simulink model "Interleaved_Boost_Thevenin_Full_Control_ForDesign"  (R2024b)
settings: Solver=FixedStepAuto  StartTime=0.0  StopTime=5  MaxStep=1e-6  RelTol=1e-3
libraries: spsSeriesRLCBranchLib x6, spsCurrentMeasurementLib x5, spsMosfetLib x3, spsDiodeLib x2, spsVoltageMeasurementLib x2, spsDCVoltageSourceLib x1, sps_lib x1
settings Model: Creator=Parti  LastModifiedBy=Eng.Abd-Elrhman Saad

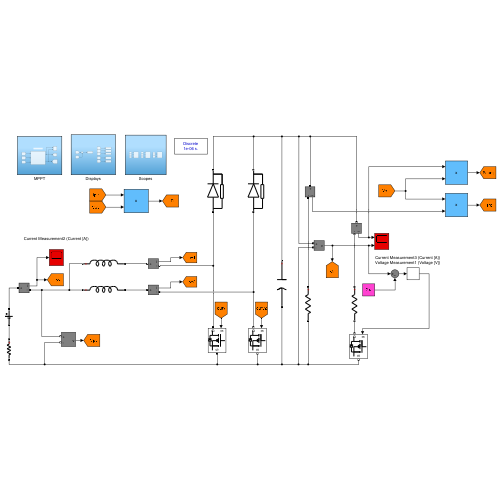
[thumbnail: Simulink's stored preview of the top-level diagram]
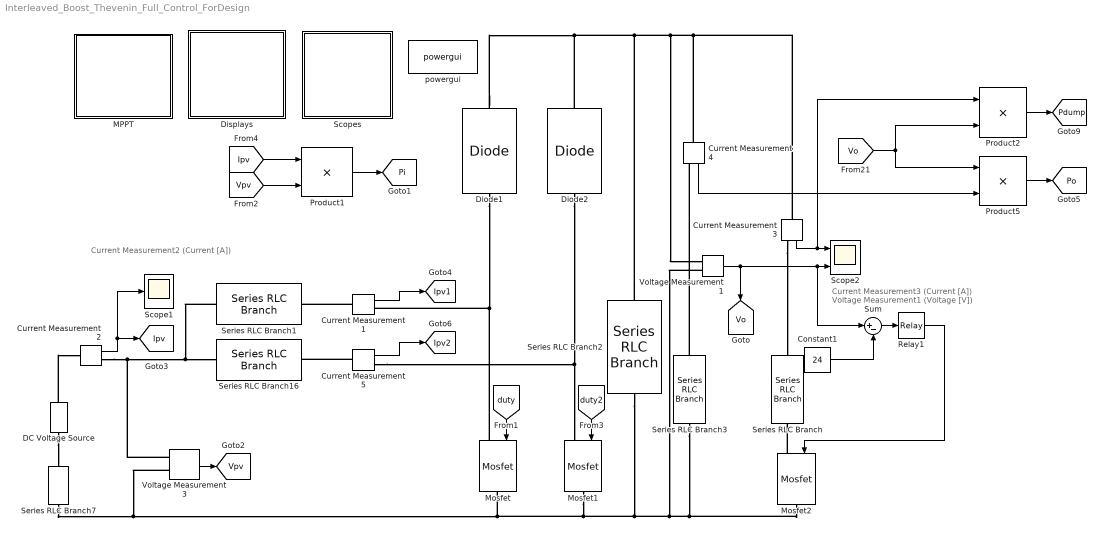
== system Interleaved_Boost_Thevenin_Full_Control_ForDesign ==
  note: Current Measurement2 (Current [A])
  note: Current Measurement3 (Current [A])
      | Voltage Measurement1 (Voltage [V])
  Constant1 : Constant  Value=24
  Current Measurement{1..5} (5 alike) : spsCurrentMeasurementLib/Current Measurement  PhasorSimulation=off  OutputType=Complex  PSBequivalent=0
  DC Voltage Source : spsDCVoltageSourceLib/DC Voltage Source  Amplitude=12  Measurements=None
  Diode1 : spsDiodeLib/Diode  Ron=0.001  Lon=0  Vf=0.8  IC=0  UseSnubber=0  Rs=500  Cs=250e-9  Measurements=off
  Diode2 : spsDiodeLib/Diode  Ron=0.001  Lon=0  Vf=0.8  IC=0  UseSnubber=0  Rs=500  Cs=250e-9  Measurements=off
  "Displays " : Subsystem
  MPPT : Subsystem
  Mosfet : spsMosfetLib/Mosfet  Ron=0.1  Lon=0  Rd=0.01  Vfd=0  IC=0  Rs=1e5  Cs=inf  Measurements=off
  Mosfet1 : spsMosfetLib/Mosfet  Ron=0.1  Lon=0  Rd=0.01  Vfd=0  IC=0  Rs=1e5  Cs=inf  Measurements=off
  Mosfet2 : spsMosfetLib/Mosfet  Ron=0.1  Lon=0  Rd=0.01  Vfd=0  IC=0  Rs=1e5  Cs=inf  Measurements=off
  Product1 : Product
  Product2 : Product
  Product5 : Product
  Relay1 : Relay  OnSwitchValue=0.5  OffSwitchValue=-0.5
  Scope1 : Scope
  Scope2 : Scope  NumInputPorts=2
  Scopes : Subsystem
  Series RLC Branch : spsSeriesRLCBranchLib/Series RLC Branch  LConnTagsString=__new0  RConnTagsString=__new0  BranchType=R  Resistance=57.6  Inductance=1e-3  SetiL0=off  InitialCurrent=0  Capacitance=1e-6  Setx0=off  InitialVoltage=0  Measurements=None
  Series RLC Branch1 : spsSeriesRLCBranchLib/Series RLC Branch  LConnTagsString=__new0  RConnTagsString=__new0  BranchType=L  Resistance=1  Inductance=2e-3  SetiL0=off  InitialCurrent=0  Capacitance=1000e-6  Setx0=on  InitialVoltage=100  Measurements=None
  Series RLC Branch16 : spsSeriesRLCBranchLib/Series RLC Branch  LConnTagsString=__new0  RConnTagsString=__new0  BranchType=L  Resistance=1  Inductance=2e-3  SetiL0=off  InitialCurrent=0  Capacitance=1000e-6  Setx0=on  InitialVoltage=100  Measurements=None
  Series RLC Branch2 : spsSeriesRLCBranchLib/Series RLC Branch  LConnTagsString=__new0  RConnTagsString=__new0  BranchType=C  Resistance=1  Inductance=1e-3  SetiL0=off  InitialCurrent=0  Capacitance=2e-3  Setx0=off  InitialVoltage=24  Measurements=None
  Series RLC Branch3 : spsSeriesRLCBranchLib/Series RLC Branch  LConnTagsString=__new0  RConnTagsString=__new0  BranchType=R  Resistance=220  Inductance=1e-3  SetiL0=off  InitialCurrent=0  Capacitance=1e-6  Setx0=off  InitialVoltage=0  Measurements=None
  Series RLC Branch7 : spsSeriesRLCBranchLib/Series RLC Branch  LConnTagsString=__new0  RConnTagsString=__new0  BranchType=R  Resistance=7  Inductance=1e-3  SetiL0=off  InitialCurrent=0  Capacitance=1e-6  Setx0=off  InitialVoltage=0  Measurements=None
  Sum : Sum  Inputs=|+-
  Voltage Measurement1 : spsVoltageMeasurementLib/Voltage Measurement  PhasorSimulation=off  OutputType=Complex  PSBequivalent=0
  Voltage Measurement3 : spsVoltageMeasurementLib/Voltage Measurement  PhasorSimulation=off  OutputType=Complex  PSBequivalent=0
  powergui : sps_lib/powergui  Priority=1  SimulationMode=Discrete  SampleTime=1e-6  frequency=60  Iterations=50  frequencyindice=0  Pbase=100e6  ErrMax=1e-4  UnitsV=kV  UnitsW=MW  buscounter=0  FunctionMessages=off  echomessages=off  EnableUseOfTLC=off  CurrentSourceSwitches=off  DisableSnubberDevices=off  DisableRonSwitches=off  DisableVfSwitches=off  DisplayEquations=off  AutomaticDiscreteSolvers=off  SolverType=Tustin/Backward Euler (TBE)  Interpol=off  ExternalGateDelay=off  methode=off  Ts=100  x0status=blocks  SPID=on  SwTol=0  HookPort=off  NonlinearTolerance=1e-4  nMaxIteration=100  ContinueOnMaxIteration=off  RestoreLinks=warning  ResistiveCurrentMeasurement=off  Frange=[0:2:500]  Ylog=off  Xlog=on  ShowGrid=off  save=off  variable=ZData  structure=0  ZoomFFT=off  StartTime=0.0  cycles=1  DisplayStyle=1  fundamental=60  FreqAxis=off  MaxFrequency=1000  frequencyindicesteady=1  RmsSteady=1  display=off
  tag scope: Ipv1=global, Ipv2=global, Ipv=global, Pdump=global, Pi=global, Po=global, Vo=global, Vpv=global
  wires:
  Current Measurement3/1 -> Product2/1, Scope2/1
  Voltage Measurement1/1 -> Scope2/2, Sum/1, [Vo]
  Current Measurement1/1 -> [Ipv1]
  Current Measurement5/1 -> [Ipv2]
  Constant1/1 -> Sum/2
  Sum/1 -> Relay1/1
  Relay1/1 -> Mosfet2/1
  [duty] -> Mosfet/1
  Voltage Measurement3/1 -> [Vpv]
  Current Measurement2/1 -> Scope1/1, [Ipv]
  [Ipv] -> Product1/1
  Product5/1 -> [Po]
  [Vpv] -> Product1/2
  Product1/1 -> [Pi]
  Current Measurement4/1 -> Product5/2
  Product2/1 -> [Pdump]
  [Vo] -> Product5/1, Product2/2
  [duty2] -> Mosfet1/1
  connections:
  Current Measurement5/LConn1 -- Series RLC Branch16/RConn1
  Diode1/RConn1 -- Current Measurement4/LConn1 -- Current Measurement3/LConn1 -- Voltage Measurement1/LConn1 -- Series RLC Branch2/LConn1 -- Diode2/RConn1
  Series RLC Branch2/RConn1 -- Mosfet2/RConn1 -- Series RLC Branch3/RConn1 -- Voltage Measurement1/LConn2 -- Mosfet1/RConn1 -- Series RLC Branch7/RConn1 -- Voltage Measurement3/LConn2 -- Mosfet/RConn1
  DC Voltage Source/RConn1 -- Current Measurement2/LConn1
  Current Measurement2/RConn1 -- Voltage Measurement3/LConn1 -- Series RLC Branch1/LConn1 -- Series RLC Branch16/LConn1
  Current Measurement3/RConn1 -- Series RLC Branch/LConn1
  Diode2/LConn1 -- Current Measurement5/RConn1 -- Mosfet1/LConn1
  Current Measurement1/LConn1 -- Series RLC Branch1/RConn1
  Diode1/LConn1 -- Mosfet/LConn1 -- Current Measurement1/RConn1
  Mosfet2/LConn1 -- Series RLC Branch/RConn1
  DC Voltage Source/LConn1 -- Series RLC Branch7/LConn1
  Series RLC Branch3/LConn1 -- Current Measurement4/RConn1

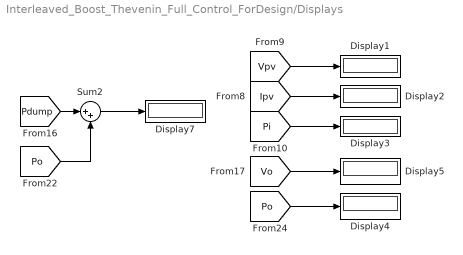
== system Interleaved_Boost_Thevenin_Full_Control_ForDesign/Displays  ==
  Display{1..5,7} (6 alike) : Display
  Sum2 : Sum  Inputs=|++
  wires:
  Sum2/1 -> Display7/1
  [Pi] -> Display3/1
  [Pdump] -> Sum2/1
  [Po] -> Display4/1
  [Po] -> Sum2/2
  [Ipv] -> Display2/1
  [Vpv] -> Display1/1
  [Vo] -> Display5/1

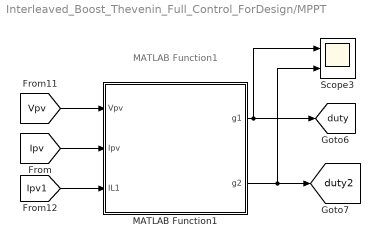
== system Interleaved_Boost_Thevenin_Full_Control_ForDesign/MPPT ==
  note: MATLAB Function1
  MATLAB Function1 : MATLAB Function  TreatAsAtomicUnit=on
  Scope3 : Scope  NumInputPorts=2
  tag scope: duty2=global, duty=global
  wires:
  [Ipv1] -> MATLAB Function1/3(IL1)
  [Ipv] -> MATLAB Function1/2(Ipv)
  MATLAB Function1/1(g1) -> Scope3/1, [duty]
  MATLAB Function1/2(g2) -> Scope3/2, [duty2]
  [Vpv] -> MATLAB Function1/1(Vpv)

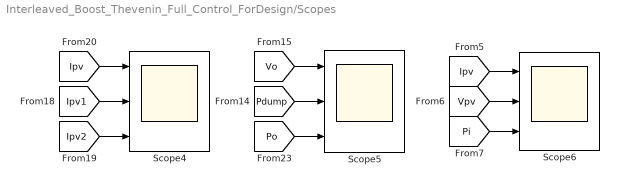
== system Interleaved_Boost_Thevenin_Full_Control_ForDesign/Scopes ==
  Scope4 : Scope  NumInputPorts=3
  Scope5 : Scope  NumInputPorts=3
  Scope6 : Scope  NumInputPorts=3
  wires:
  [Ipv1] -> Scope4/2
  [Vo] -> Scope5/1
  [Po] -> Scope5/3
  [Pdump] -> Scope5/2
  [Ipv] -> Scope6/1
  [Ipv2] -> Scope4/3
  [Ipv] -> Scope4/1
  [Pi] -> Scope6/3
  [Vpv] -> Scope6/2

== matlab function Interleaved_Boost_Thevenin_Full_Control_ForDesign/MPPT/MATLAB Function1 ==
  data: Vpv input; Ipv input; g1 output; IL1 input; g2 output
function [g1, g2] = mppt_controller_pwm(Vpv, Ipv, IL1)
    persistent V_target Pmax Vbest mode timer;
    persistent err_int_v err_int_i t;
    
    Ts = 1e-6;      
    fsw = 10e3;     
    Tsw = 1/fsw;
    
    if isempty(V_target)
        V_target = Vpv; 
        Pmax = 0;
        Vbest = Vpv;
        mode = 0;
        timer = 0;
        err_int_v = 0;
        err_int_i = 0;
        t = 0;
    end
    
    % ===== Internal Calculation of IL2 =====
    % Based on the nodal equation: Ipv = IL1 + IL2
    IL2 = Ipv - IL1; 
    
    % ===== MPPT Logic (Scanning) =====
    Ppv = Vpv * Ipv;
    V_ramp_rate = 200; 
    
    switch mode
        case 0 % Initialization
            V_target = Vpv;
            Pmax = 0;
            mode = 1;
            
        case 1 % Scanning Downward
            if Ppv > Pmax
                Pmax = Ppv;
                Vbest = Vpv;
            end
            V_target = V_target - (V_ramp_rate * Ts);
            % Stop scan at 50% of starting voltage
            if V_target <= 0.5 * Vbest 
                mode = 2;
            end
            
        case 2 % Return to Vbest
            V_target = Vbest;
            mode = 3;
            timer = 0;
            
        case 3 % Hold and Dwell
            timer = timer + Ts;
            if timer >= 5 
                mode = 0; % Restart scan
            end
    end
    
    % ===== Outer Loop: Voltage Control (Vpv -> Iref) =====
    err_v = Vpv - V_target; 
    
    Kp_v = 1.5; 
    Ki_v = 80;
    
    err_int_v = err_int_v + err_v * Ts;
    err_int_v = max(min(err_int_v, 0.5), -0.5); 
    
    Iref_total = Kp_v * err_v + Ki_v * err_int_v; 
    Iref_total = max(min(Iref_total, 20), 0); 
    
    % ===== Inner Loop: Current Control (Iref -> Duty) =====
    Iref_phase = 0.5 * Iref_total;
    
    err_i1 = Iref_phase - IL1;
    err_i2 = Iref_phase - IL2;
    
    Kp_i = 1; 
    Ki_i = 100;
    
    err_int_i = err_int_i + (err_i1 + err_i2) * Ts; 
    err_int_i = max(min(err_int_i, 10), -10);
    
    % Duty cycle calculation
    duty1 = Kp_i * err_i1 + Ki_i * err_int_i;
    duty2 = Kp_i * err_i2 + Ki_i * err_int_i;
    
    % Safety Clamps
    duty1 = max(min(duty1, 0.9), 0.1);
    duty2 = max(min(duty2, 0.9), 0.1);
    
    % ===== PWM Generation (180 deg Phase Shift) =====
    t = t + Ts;
    if t >= Tsw, t = 0; end 
    
    carrier1 = t / Tsw;
    carrier2 = mod(t + Tsw/2, Tsw) / Tsw;
    
    % ===== Gate signals =====
    g1 = (duty1 > carrier1);
    g2 = (duty2 > carrier2);
end
